simulink model "Diagnostic"  (R2024a)
settings: Solver=FixedStepDiscrete  StartTime=0.0  StopTime=10.0  RelTol=1e-3  EnableMultiTasking=on
undefined symbols (not defined in the file): DIAG_DEBOUNCE_CNT, DiagEventStatus_T, RadarStatus_T, SignalStatus_T
libraries: simulink x12
settings Model: DataDictionary=bsd.sldd  Creator=pc  LastModifiedBy=pc
settings OptimizationCC: DefaultParameterBehavior=Inlined  UseDivisionForNetSlopeComputation=on  EnhancedBackFolding=on  PassReuseOutputArgsAs=Individual arguments  ZeroExternalMemoryAtStartup=off  ZeroInternalMemoryAtStartup=off  OptimizeBlockOrder=speed  DifferentSizesBufferReuse=on  OptimizationCustomize=off  EfficientTunableParamExpr=on
settings DebuggingCC: ParameterTunabilityLossMsg=error
settings SFSimCC: MATLABDynamicMemAlloc=off
settings RTWCC: Description=AUTOSAR  SystemTargetFile=autosar.tlc  GenCodeOnly=on  TemplateMakefile=ert_default_tmf  DataTypeReplacement=CDataTypesFixedWidth
settings CodeAppCC: ForceParamTrailComments=on  IgnoreCustomStorageClasses=off  OperatorAnnotations=on  SimulinkDataObjDesc=on  SFDataObjDesc=on  InsertBlockDesc=on
settings STFCustomTargetCC: MultiwordLength=256  ParMdlRefBuildCompliant=on  CompOptLevelCompliant=on  IncludeMdlTerminateFcn=off  CombineOutputUpdateFcns=on  SuppressErrorStatus=on  ERTCustomFileBanners=on  SupportNonFinite=off  SupportComplex=off  SupportContinuousTime=off  SupportNonInlinedSFcns=off  RemoveResetFunc=on  MATLABClassNameForMDSCustomization=Simulink.SoftwareTarget.ERTCustomization  AutosarCompliant=on  GRTInterface=off  LookupTableObjectStructAxisOrder=2,1,3,4,...  LUTObjectStructOrderEvenSpacing=Size,Table,Breakpoints  SystemTargetFile=autosar.tlc
settings ERTTargetCC: TargetLangStandard=C99 (ISO)  ConcurrentExecutionCompliant=off  IncludeMdlTerminateFcn=off  SuppressErrorStatus=on  SupportNonFinite=off  SupportComplex=off  ModelStepFunctionPrototypeControlCompliant=off  CPPClassGenCompliant=off  AutosarCompliant=on  LookupTableObjectStructAxisOrder=2,1,3,4,...  LUTObjectStructOrderEvenSpacing=Size,Table,Breakpoints  InlinedParameterPlacement=NonHierarchical  ERTCustomFileTemplate=example_file_process.tlc  BooleanTrueId=TRUE  BooleanFalseId=FALSE

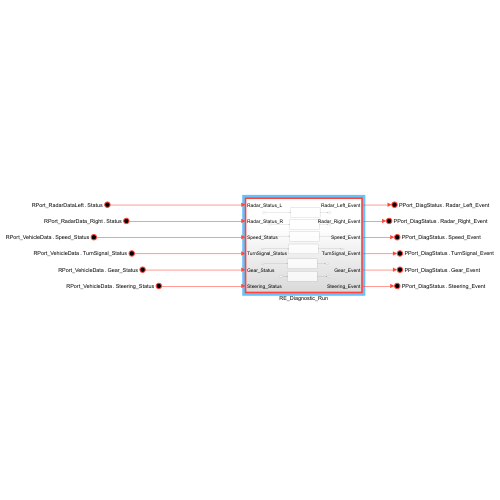
[thumbnail: Simulink's stored preview of the top-level diagram]
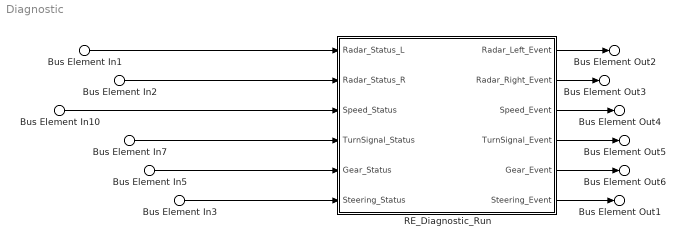
== system Diagnostic ==
  Bus Element In3 : Inport  PortName=RPort_VehicleData  Element=Steering_Status
  Bus Element In5 : Inport  PortName=RPort_VehicleData  Element=Gear_Status
  Bus Element In7 : Inport  PortName=RPort_VehicleData  Element=TurnSignal_Status
  Bus Element In10 : Inport  PortName=RPort_VehicleData  Element=Speed_Status
  Bus Element In2 : Inport  Port=2  PortName=RPort_RadarData_Right  Element=Status
  Bus Element In1 : Inport  Port=3  PortName=RPort_RadarDataLeft  Element=Status
  RE_Diagnostic_Run : Subsystem  TreatAsAtomicUnit=on
  Bus Element Out1 : Outport  PortName=PPort_DiagStatus  Element=Steering_Event
  Bus Element Out2 : Outport  PortName=PPort_DiagStatus  Element=Radar_Left_Event
  Bus Element Out3 : Outport  PortName=PPort_DiagStatus  Element=Radar_Right_Event
  Bus Element Out4 : Outport  PortName=PPort_DiagStatus  Element=Speed_Event
  Bus Element Out5 : Outport  PortName=PPort_DiagStatus  Element=TurnSignal_Event
  Bus Element Out6 : Outport  PortName=PPort_DiagStatus  Element=Gear_Event
  wires:
  Bus Element In1/1 -> RE_Diagnostic_Run/1(Radar_Status_L)
  Bus Element In2/1 -> RE_Diagnostic_Run/2(Radar_Status_R)
  Bus Element In10/1 -> RE_Diagnostic_Run/3(Speed_Status)
  Bus Element In7/1 -> RE_Diagnostic_Run/4(TurnSignal_Status)
  Bus Element In5/1 -> RE_Diagnostic_Run/5(Gear_Status)
  Bus Element In3/1 -> RE_Diagnostic_Run/6(Steering_Status)
  RE_Diagnostic_Run/1(Radar_Left_Event) -> Bus Element Out2/1
  RE_Diagnostic_Run/2(Radar_Right_Event) -> Bus Element Out3/1
  RE_Diagnostic_Run/3(Speed_Event) -> Bus Element Out4/1
  RE_Diagnostic_Run/4(TurnSignal_Event) -> Bus Element Out5/1
  RE_Diagnostic_Run/5(Gear_Event) -> Bus Element Out6/1
  RE_Diagnostic_Run/6(Steering_Event) -> Bus Element Out1/1

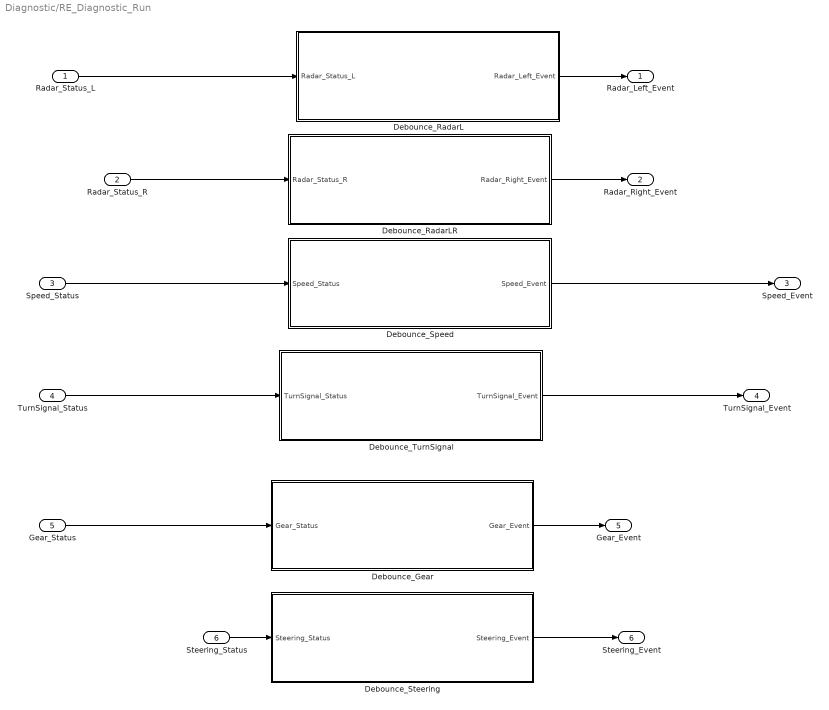
== system Diagnostic/RE_Diagnostic_Run ==
  Radar_Status_L : Inport  OutDataTypeStr=Enum: RadarStatus_T
  Radar_Status_R : Inport  Port=2  OutDataTypeStr=Enum: RadarStatus_T
  Speed_Status : Inport  Port=3  OutDataTypeStr=Enum: SignalStatus_T
  TurnSignal_Status : Inport  Port=4  OutDataTypeStr=Enum: SignalStatus_T
  Gear_Status : Inport  Port=5  OutDataTypeStr=Enum: SignalStatus_T
  Steering_Status : Inport  Port=6  OutDataTypeStr=Enum: SignalStatus_T
  Debounce_Gear : Subsystem
  Debounce_RadarL : Subsystem
  Debounce_RadarLR : Subsystem
  Debounce_Speed : Subsystem
  Debounce_Steering : Subsystem
  Debounce_TurnSignal : Subsystem
  Radar_Left_Event : Outport  OutDataTypeStr=Enum: DiagEventStatus_T
  Radar_Right_Event : Outport  Port=2  OutDataTypeStr=Enum: DiagEventStatus_T
  Speed_Event : Outport  Port=3  OutDataTypeStr=Enum: DiagEventStatus_T
  TurnSignal_Event : Outport  Port=4  OutDataTypeStr=Enum: DiagEventStatus_T
  Gear_Event : Outport  Port=5  OutDataTypeStr=Enum: DiagEventStatus_T
  Steering_Event : Outport  Port=6  OutDataTypeStr=Enum: DiagEventStatus_T
  wires:
  Debounce_Steering/1(Steering_Event) -> Steering_Event/1
  Debounce_Gear/1(Gear_Event) -> Gear_Event/1
  Debounce_RadarL/1(Radar_Left_Event) -> Radar_Left_Event/1
  Debounce_Speed/1(Speed_Event) -> Speed_Event/1
  Debounce_TurnSignal/1(TurnSignal_Event) -> TurnSignal_Event/1
  Debounce_RadarLR/1(Radar_Right_Event) -> Radar_Right_Event/1
  Radar_Status_L/1 -> Debounce_RadarL/1(Radar_Status_L)
  Radar_Status_R/1 -> Debounce_RadarLR/1(Radar_Status_R)
  Speed_Status/1 -> Debounce_Speed/1(Speed_Status)
  TurnSignal_Status/1 -> Debounce_TurnSignal/1(TurnSignal_Status)
  Gear_Status/1 -> Debounce_Gear/1(Gear_Status)
  Steering_Status/1 -> Debounce_Steering/1(Steering_Status)

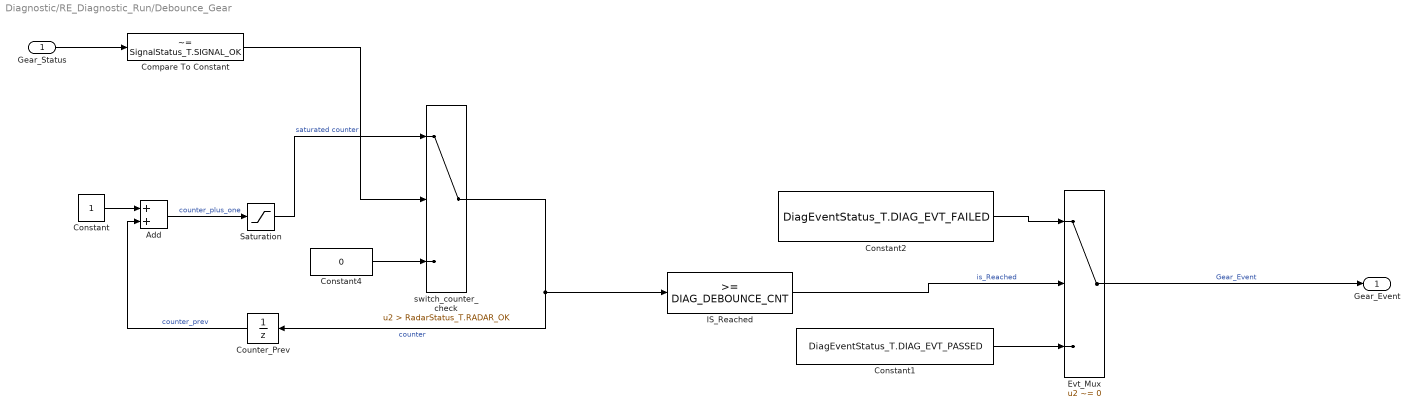
== system Diagnostic/RE_Diagnostic_Run/Debounce_Gear ==
  Gear_Status : Inport
  Add : Sum  OutDataTypeStr=uint8
  Compare To Constant : simulink/Logic and Bit Operations/Compare To Constant  relop=~=  const=SignalStatus_T.SIGNAL_OK  OutDataTypeStr=boolean
  Constant : Constant  OutDataTypeStr=uint8
  Constant1 : Constant  Value=DiagEventStatus_T.DIAG_EVT_PASSED  OutDataTypeStr=Enum: DiagEventStatus_T
  Constant2 : Constant  Value=DiagEventStatus_T.DIAG_EVT_FAILED  OutDataTypeStr=Enum: DiagEventStatus_T
  Constant4 : Constant  Value=0
  Counter_Prev : UnitDelay  SampleTime=-1  HasFrameUpgradeWarning=on
  Evt_Mux : Switch  Criteria=u2 ~= 0  OutDataTypeStr=Enum: DiagEventStatus_T  SaturateOnIntegerOverflow=off  InputSameDT=off
  IS_Reached : simulink/Logic and Bit Operations/Compare To Constant  relop=>=  const=DIAG_DEBOUNCE_CNT  OutDataTypeStr=boolean
  Saturation : Saturate  UpperLimit=DIAG_DEBOUNCE_CNT  LowerLimit=0  OutDataTypeStr=uint8
  switch_counter_check : Switch  Criteria=u2 > Threshold  Threshold=RadarStatus_T.RADAR_OK  OutDataTypeStr=uint8  SaturateOnIntegerOverflow=off  InputSameDT=off
  Gear_Event : Outport  OutDataTypeStr=Enum: DiagEventStatus_T
  wires:
  IS_Reached/1 -> Evt_Mux/2  "is_Reached"
  Constant4/1 -> switch_counter_check/3
  Evt_Mux/1 -> Gear_Event/1  "Gear_Event"
  Constant2/1 -> Evt_Mux/1
  Gear_Status/1 -> Compare To Constant/1
  switch_counter_check/1 -> IS_Reached/1, Counter_Prev/1  "counter"
  Constant/1 -> Add/1
  Saturation/1 -> switch_counter_check/1  "saturated counter"
  Counter_Prev/1 -> Add/2  "counter_prev"
  Add/1 -> Saturation/1  "counter_plus_one"
  Constant1/1 -> Evt_Mux/3
  Compare To Constant/1 -> switch_counter_check/2

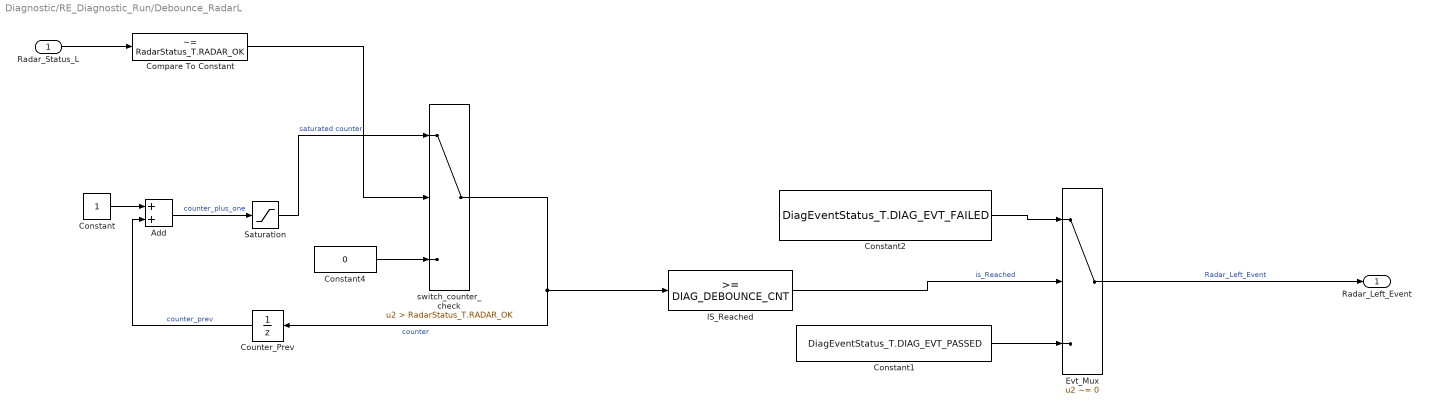
== system Diagnostic/RE_Diagnostic_Run/Debounce_RadarL ==
  Radar_Status_L : Inport
  Add : Sum  OutDataTypeStr=uint8
  Compare To Constant : simulink/Logic and Bit Operations/Compare To Constant  relop=~=  const=RadarStatus_T.RADAR_OK  OutDataTypeStr=boolean
  Constant : Constant  OutDataTypeStr=uint8
  Constant1 : Constant  Value=DiagEventStatus_T.DIAG_EVT_PASSED  OutDataTypeStr=Enum: DiagEventStatus_T
  Constant2 : Constant  Value=DiagEventStatus_T.DIAG_EVT_FAILED  OutDataTypeStr=Enum: DiagEventStatus_T
  Constant4 : Constant  Value=0
  Counter_Prev : UnitDelay  SampleTime=-1  HasFrameUpgradeWarning=on
  Evt_Mux : Switch  Criteria=u2 ~= 0  OutDataTypeStr=Enum: DiagEventStatus_T  SaturateOnIntegerOverflow=off  InputSameDT=off
  IS_Reached : simulink/Logic and Bit Operations/Compare To Constant  relop=>=  const=DIAG_DEBOUNCE_CNT  OutDataTypeStr=boolean
  Saturation : Saturate  UpperLimit=DIAG_DEBOUNCE_CNT  LowerLimit=0  OutDataTypeStr=uint8
  switch_counter_check : Switch  Criteria=u2 > Threshold  Threshold=RadarStatus_T.RADAR_OK  OutDataTypeStr=uint8  SaturateOnIntegerOverflow=off  InputSameDT=off
  Radar_Left_Event : Outport  OutDataTypeStr=Enum: DiagEventStatus_T
  wires:
  Constant/1 -> Add/1
  Saturation/1 -> switch_counter_check/1  "saturated counter"
  Constant1/1 -> Evt_Mux/3
  Evt_Mux/1 -> Radar_Left_Event/1  "Radar_Left_Event"
  IS_Reached/1 -> Evt_Mux/2  "is_Reached"
  Constant2/1 -> Evt_Mux/1
  Constant4/1 -> switch_counter_check/3
  Counter_Prev/1 -> Add/2  "counter_prev"
  Add/1 -> Saturation/1  "counter_plus_one"
  Radar_Status_L/1 -> Compare To Constant/1
  switch_counter_check/1 -> Counter_Prev/1, IS_Reached/1  "counter"
  Compare To Constant/1 -> switch_counter_check/2

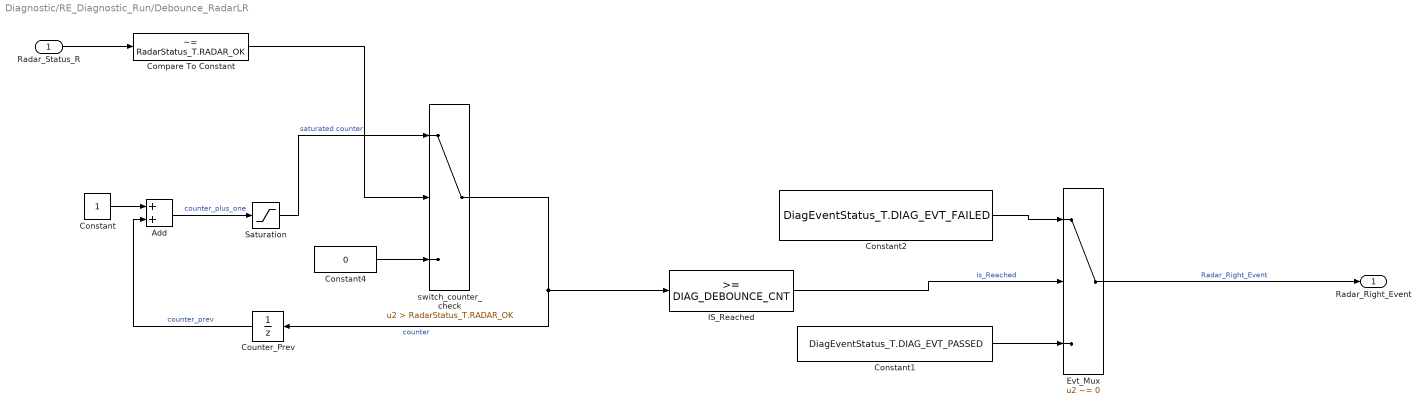
== system Diagnostic/RE_Diagnostic_Run/Debounce_RadarLR ==
  Radar_Status_R : Inport
  Add : Sum  OutDataTypeStr=uint8
  Compare To Constant : simulink/Logic and Bit Operations/Compare To Constant  relop=~=  const=RadarStatus_T.RADAR_OK  OutDataTypeStr=boolean
  Constant : Constant  OutDataTypeStr=uint8
  Constant1 : Constant  Value=DiagEventStatus_T.DIAG_EVT_PASSED  OutDataTypeStr=Enum: DiagEventStatus_T
  Constant2 : Constant  Value=DiagEventStatus_T.DIAG_EVT_FAILED  OutDataTypeStr=Enum: DiagEventStatus_T
  Constant4 : Constant  Value=0
  Counter_Prev : UnitDelay  SampleTime=-1  HasFrameUpgradeWarning=on
  Evt_Mux : Switch  Criteria=u2 ~= 0  OutDataTypeStr=Enum: DiagEventStatus_T  SaturateOnIntegerOverflow=off  InputSameDT=off
  IS_Reached : simulink/Logic and Bit Operations/Compare To Constant  relop=>=  const=DIAG_DEBOUNCE_CNT  OutDataTypeStr=boolean
  Saturation : Saturate  UpperLimit=DIAG_DEBOUNCE_CNT  LowerLimit=0  OutDataTypeStr=uint8
  switch_counter_check : Switch  Criteria=u2 > Threshold  Threshold=RadarStatus_T.RADAR_OK  OutDataTypeStr=uint8  SaturateOnIntegerOverflow=off  InputSameDT=off
  Radar_Right_Event : Outport  OutDataTypeStr=Enum: DiagEventStatus_T
  wires:
  Compare To Constant/1 -> switch_counter_check/2
  Constant1/1 -> Evt_Mux/3
  Add/1 -> Saturation/1  "counter_plus_one"
  Counter_Prev/1 -> Add/2  "counter_prev"
  Saturation/1 -> switch_counter_check/1  "saturated counter"
  Constant/1 -> Add/1
  switch_counter_check/1 -> Counter_Prev/1, IS_Reached/1  "counter"
  Radar_Status_R/1 -> Compare To Constant/1
  Constant2/1 -> Evt_Mux/1
  Evt_Mux/1 -> Radar_Right_Event/1  "Radar_Right_Event"
  Constant4/1 -> switch_counter_check/3
  IS_Reached/1 -> Evt_Mux/2  "is_Reached"

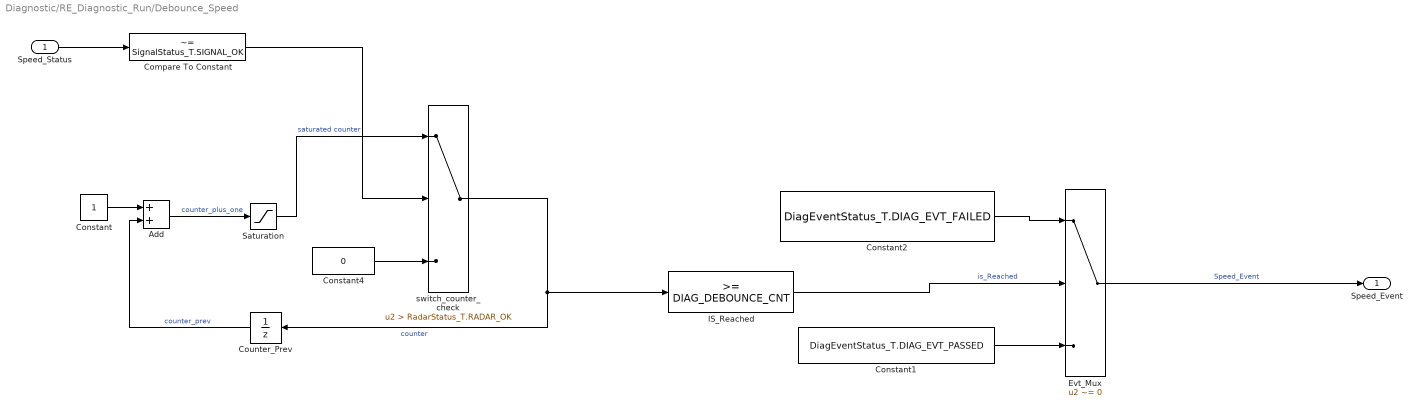
== system Diagnostic/RE_Diagnostic_Run/Debounce_Speed ==
  Speed_Status : Inport
  Add : Sum  OutDataTypeStr=uint8
  Compare To Constant : simulink/Logic and Bit Operations/Compare To Constant  relop=~=  const=SignalStatus_T.SIGNAL_OK  OutDataTypeStr=boolean
  Constant : Constant  OutDataTypeStr=uint8
  Constant1 : Constant  Value=DiagEventStatus_T.DIAG_EVT_PASSED  OutDataTypeStr=Enum: DiagEventStatus_T
  Constant2 : Constant  Value=DiagEventStatus_T.DIAG_EVT_FAILED  OutDataTypeStr=Enum: DiagEventStatus_T
  Constant4 : Constant  Value=0
  Counter_Prev : UnitDelay  SampleTime=-1  HasFrameUpgradeWarning=on
  Evt_Mux : Switch  Criteria=u2 ~= 0  OutDataTypeStr=Enum: DiagEventStatus_T  SaturateOnIntegerOverflow=off  InputSameDT=off
  IS_Reached : simulink/Logic and Bit Operations/Compare To Constant  relop=>=  const=DIAG_DEBOUNCE_CNT  OutDataTypeStr=boolean
  Saturation : Saturate  UpperLimit=DIAG_DEBOUNCE_CNT  LowerLimit=0  OutDataTypeStr=uint8
  switch_counter_check : Switch  Criteria=u2 > Threshold  Threshold=RadarStatus_T.RADAR_OK  OutDataTypeStr=uint8  SaturateOnIntegerOverflow=off  InputSameDT=off
  Speed_Event : Outport  OutDataTypeStr=Enum: DiagEventStatus_T
  wires:
  IS_Reached/1 -> Evt_Mux/2  "is_Reached"
  Constant4/1 -> switch_counter_check/3
  Evt_Mux/1 -> Speed_Event/1  "Speed_Event"
  Constant2/1 -> Evt_Mux/1
  Speed_Status/1 -> Compare To Constant/1
  switch_counter_check/1 -> IS_Reached/1, Counter_Prev/1  "counter"
  Constant/1 -> Add/1
  Saturation/1 -> switch_counter_check/1  "saturated counter"
  Counter_Prev/1 -> Add/2  "counter_prev"
  Add/1 -> Saturation/1  "counter_plus_one"
  Constant1/1 -> Evt_Mux/3
  Compare To Constant/1 -> switch_counter_check/2

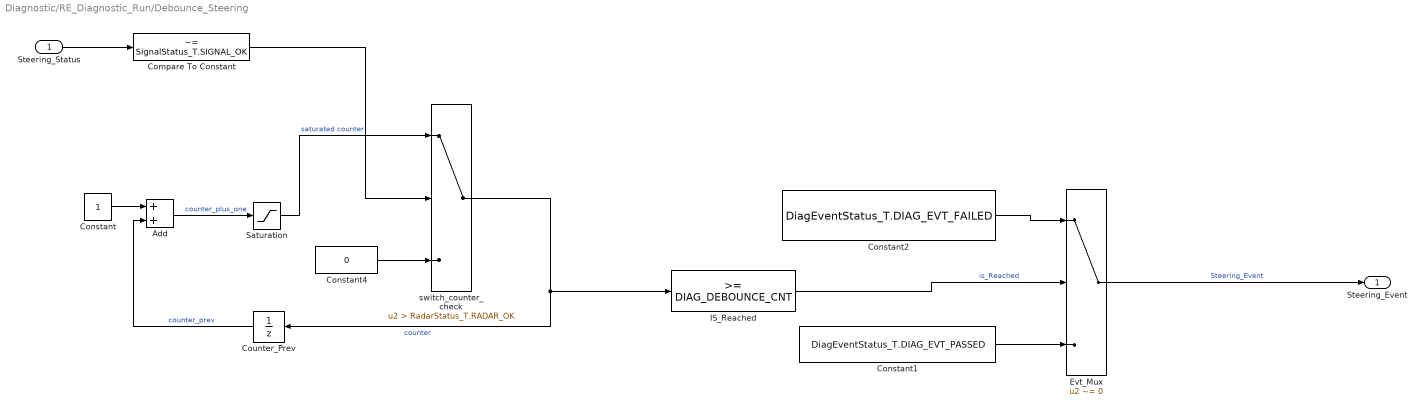
== system Diagnostic/RE_Diagnostic_Run/Debounce_Steering ==
  Steering_Status : Inport
  Add : Sum  OutDataTypeStr=uint8
  Compare To Constant : simulink/Logic and Bit Operations/Compare To Constant  relop=~=  const=SignalStatus_T.SIGNAL_OK  OutDataTypeStr=boolean
  Constant : Constant  OutDataTypeStr=uint8
  Constant1 : Constant  Value=DiagEventStatus_T.DIAG_EVT_PASSED  OutDataTypeStr=Enum: DiagEventStatus_T
  Constant2 : Constant  Value=DiagEventStatus_T.DIAG_EVT_FAILED  OutDataTypeStr=Enum: DiagEventStatus_T
  Constant4 : Constant  Value=0
  Counter_Prev : UnitDelay  SampleTime=-1  HasFrameUpgradeWarning=on
  Evt_Mux : Switch  Criteria=u2 ~= 0  OutDataTypeStr=Enum: DiagEventStatus_T  SaturateOnIntegerOverflow=off  InputSameDT=off
  IS_Reached : simulink/Logic and Bit Operations/Compare To Constant  relop=>=  const=DIAG_DEBOUNCE_CNT  OutDataTypeStr=boolean
  Saturation : Saturate  UpperLimit=DIAG_DEBOUNCE_CNT  LowerLimit=0  OutDataTypeStr=uint8
  switch_counter_check : Switch  Criteria=u2 > Threshold  Threshold=RadarStatus_T.RADAR_OK  OutDataTypeStr=uint8  SaturateOnIntegerOverflow=off  InputSameDT=off
  Steering_Event : Outport  OutDataTypeStr=Enum: DiagEventStatus_T
  wires:
  Compare To Constant/1 -> switch_counter_check/2
  Constant1/1 -> Evt_Mux/3
  Add/1 -> Saturation/1  "counter_plus_one"
  Counter_Prev/1 -> Add/2  "counter_prev"
  Saturation/1 -> switch_counter_check/1  "saturated counter"
  Constant/1 -> Add/1
  switch_counter_check/1 -> Counter_Prev/1, IS_Reached/1  "counter"
  Steering_Status/1 -> Compare To Constant/1
  Constant2/1 -> Evt_Mux/1
  Evt_Mux/1 -> Steering_Event/1  "Steering_Event"
  Constant4/1 -> switch_counter_check/3
  IS_Reached/1 -> Evt_Mux/2  "is_Reached"

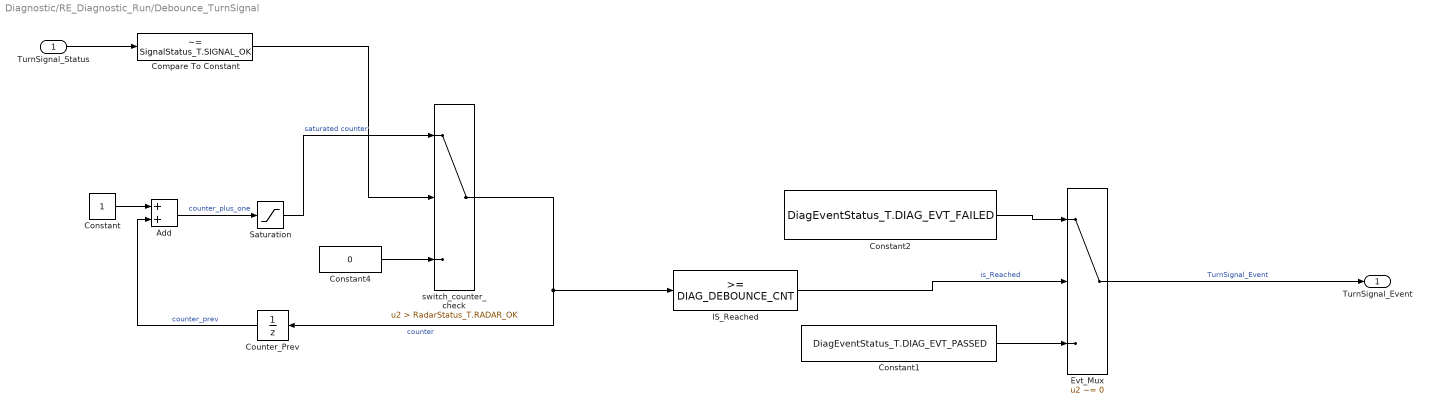
== system Diagnostic/RE_Diagnostic_Run/Debounce_TurnSignal ==
  TurnSignal_Status : Inport
  Add : Sum  OutDataTypeStr=uint8
  Compare To Constant : simulink/Logic and Bit Operations/Compare To Constant  relop=~=  const=SignalStatus_T.SIGNAL_OK  OutDataTypeStr=boolean
  Constant : Constant  OutDataTypeStr=uint8
  Constant1 : Constant  Value=DiagEventStatus_T.DIAG_EVT_PASSED  OutDataTypeStr=Enum: DiagEventStatus_T
  Constant2 : Constant  Value=DiagEventStatus_T.DIAG_EVT_FAILED  OutDataTypeStr=Enum: DiagEventStatus_T
  Constant4 : Constant  Value=0
  Counter_Prev : UnitDelay  SampleTime=-1  HasFrameUpgradeWarning=on
  Evt_Mux : Switch  Criteria=u2 ~= 0  OutDataTypeStr=Enum: DiagEventStatus_T  SaturateOnIntegerOverflow=off  InputSameDT=off
  IS_Reached : simulink/Logic and Bit Operations/Compare To Constant  relop=>=  const=DIAG_DEBOUNCE_CNT  OutDataTypeStr=boolean
  Saturation : Saturate  UpperLimit=DIAG_DEBOUNCE_CNT  LowerLimit=0  OutDataTypeStr=uint8
  switch_counter_check : Switch  Criteria=u2 > Threshold  Threshold=RadarStatus_T.RADAR_OK  OutDataTypeStr=uint8  SaturateOnIntegerOverflow=off  InputSameDT=off
  TurnSignal_Event : Outport  OutDataTypeStr=Enum: DiagEventStatus_T
  wires:
  Compare To Constant/1 -> switch_counter_check/2
  Constant1/1 -> Evt_Mux/3
  Add/1 -> Saturation/1  "counter_plus_one"
  Counter_Prev/1 -> Add/2  "counter_prev"
  Saturation/1 -> switch_counter_check/1  "saturated counter"
  Constant/1 -> Add/1
  switch_counter_check/1 -> Counter_Prev/1, IS_Reached/1  "counter"
  TurnSignal_Status/1 -> Compare To Constant/1
  Constant2/1 -> Evt_Mux/1
  Evt_Mux/1 -> TurnSignal_Event/1  "TurnSignal_Event"
  Constant4/1 -> switch_counter_check/3
  IS_Reached/1 -> Evt_Mux/2  "is_Reached"
